simulink model "GHAME_Public"  (R2024a)
settings: Solver=ode8  StartTime=0.0  StopTime=Sim.simulation.duration  FixedStep=0.01  RelTol=1e-3
undefined symbols (not defined in the file): Data, DataPlant, IC, Sim, v0_BE_B
libraries: simulink_extras x8, simulink x1
(part 2 of 3)

== matlab function GHAME_Public/GHAME Airframe/Forces and Moments/PROPULSION/Subsystem/Updating mass and inertia ==
  data: IBBB output size=[3 3]; IBBBdot output; fmdot input; fmasse input; vmass output size=[1 1]; Sim parameter; stop_flag output
function [IBBB, IBBBdot, vmass, stop_flag] = mass(fmdot, fmasse, Sim)
% MASS  Vehicle mass and inertia as a function of expended fuel.
%
%   [IBBB, IBBBdot, vmass, stop_flag] = mass(fmdot, fmasse, Sim)
%
%   The inertia tensor is interpolated linearly between the full-tank and
%   empty-tank values according to the remaining fuel fraction.
%
%   Inputs
%     fmdot   [1x1]  Fuel mass flow (kg/s)
%     fmasse  [1x1]  Fuel mass expended since start (kg)
%     Sim     struct Vehicle mass and inertia data
%
%   Outputs
%     IBBB       [3x3]  Inertia tensor in body axes (kg m^2)
%     IBBBdot    [3x3]  Time derivative of the inertia tensor (kg m^2/s)
%     vmass      [1x1]  Current vehicle mass (kg)
%     stop_flag  [1x1]  True when the fuel is exhausted

%   Author:    Thomas Harald Müller
%   GitHub:    https://github.com/ThomasHaraldMueller
%   Copyright: (c) 2026 Thomas Harald Müller, Hamburg, Germany
%   Free to use and modify, provided this notice is kept and the author is credited.

%% Mass properties
fmass_init = Sim.vehicle.mass.fuel;          % Fuel on board at start
fmass_full = Sim.vehicle.mass.fuel_full;     % Fuel capacity
vmass_init = Sim.vehicle.mass.current;       % Total mass at start
IBBB0      = Sim.vehicle.inertia.IBBB0;      % Inertia with full tank
IBBB1      = Sim.vehicle.inertia.IBBB1;      % Inertia with empty tank

%% Mass update
% Expended fuel is limited to what was on board, so mass and inertia
% never drop below the empty-tank values
fmasse_c = min(fmasse, fmass_init);

vmass = vmass_init - fmasse_c;
fmass = fmass_init - fmasse_c;               % Remaining fuel

%% Inertia update
% Fuel fraction, 1 = full tank, 0 = empty tank
fuel_ratio = fmass / fmass_full;

dI   = IBBB0 - IBBB1;
IBBB = IBBB1 + dI * fuel_ratio;

% Chain rule, d(fuel_ratio)/dt = -fmdot/fmass_full. Zero once the tank is empty.
if fmass > 0
    IBBBdot = (-fmdot / fmass_full) * dI;
else
    IBBBdot = zeros(3);
end

%% Termination
stop_flag = (fmass <= 1e-6);

end

== matlab function GHAME_Public/GHAME Airframe/Environment/ENVIRONMENT/Wind and Turbulence/Wind Computation ==
  settings: updateMethod=CONTINUOUS
  data: Vwind input; VTAD input; VAEDS input; VAED output; Sim parameter; VAEDSD output
function [VAED, VAEDSD] = wind(Vwind, VTAD, VAEDS, Sim)
% WIND  Air velocity relative to Earth from mean wind and turbulence.
%
%   [VAED, VAEDSD] = wind(Vwind, VTAD, VAEDS, Sim)
%
%   The horizontal mean wind is smoothed by a first-order lag, so that
%   steps in the wind model do not excite the vehicle. Dryden turbulence
%   is added on top when enabled. The air-relative velocity of the vehicle
%   then follows as VBAD = VBED - VAED.
%
%   Inputs
%     Vwind   [2x1]  Mean wind [north; east] from HWM14 (m/s)
%     VTAD    [3x1]  Turbulence velocity in geodetic axes (m/s)
%     VAEDS   [3x1]  Smoothed mean wind, integrator state (m/s)
%     Sim     struct Mode switches and wind smoothing time constant
%
%   Outputs
%     VAED    [3x1]  Air velocity relative to Earth, geodetic axes (m/s)
%     VAEDSD  [3x1]  Derivative of the smoothed mean wind (m/s^2)
%
%   Initialize the VAEDS integrator with the initial wind to avoid a
%   start-up transient.

%   Author:    Thomas Harald Müller
%   GitHub:    https://github.com/ThomasHaraldMueller
%   Copyright: (c) 2026 Thomas Harald Müller, Hamburg, Germany
%   Free to use and modify, provided this notice is kept and the author is credited.

twind = Sim.wind.tau_smooth;        % Smoothing time constant (s)

VAED   = zeros(3, 1);
VAEDSD = zeros(3, 1);

% Mean wind, smoothed by a first-order lag
if Sim.mode.mwind > 0
    VAED_raw = [Vwind(1);           % North (meridional)
                Vwind(2);           % East (zonal)
                0];                 % Down, no vertical mean wind

    VAEDSD = (VAED_raw - VAEDS) / twind;
    VAED   = VAEDS;
end

% Dryden turbulence
if Sim.mode.mturb > 0
    VAED = VAED + VTAD;
end

end

== matlab function GHAME_Public/GHAME Airframe/Environment/ENVIRONMENT/Gravity Calculation ==
  data: SBII input; GRAVG output; Sim parameter
function GRAVG = cad_grav84(SBII, Sim)
% CAD_GRAV84  Gravitational acceleration with J2 in geocentric coordinates.
%
%   GRAVG = cad_grav84(SBII, Sim)
%
%   Uses the normalized second zonal harmonic C20 of the WGS84 field.
%   The geocentric frame G is north, east, down with the down axis pointing
%   to the Earth centre. The east component is zero for a zonal field.
%
%   Inputs
%     SBII    [3x1]  Position in inertial coordinates (m)
%     Sim     struct Earth constants (GM, semi-major axis, normalized C20 < 0)
%
%   Output
%     GRAVG   [3x1]  Gravitational acceleration in geocentric axes (m/s^2)

%   Author:    Thomas Harald Müller
%   GitHub:    https://github.com/ThomasHaraldMueller
%   Copyright: (c) 2026 Thomas Harald Müller, Hamburg, Germany
%   Free to use and modify, provided this notice is kept and the author is credited.

GM  = Sim.earth.GM;
a   = Sim.earth.SMAJOR_AXIS;
C20 = Sim.earth.C20;

r    = norm(SBII);
latc = asin(SBII(3) / r);           % Geocentric latitude
slat = sin(latc);
clat = cos(latc);

g0 = GM / r^2;                      % Point-mass gravity
k  = sqrt(5) * C20 * (a / r)^2;     % J2 scaling, negative for C20 < 0

% Gradient of V = GM/r * (1 + C20*(a/r)^2 * sqrt(5)/2 * (3*sin(lat)^2 - 1))
GRAVG = [ 3 * g0 * k * slat * clat;                 % North (towards equator)
          0;                                        % East
          g0 * (1 + 1.5 * k * (3 * slat^2 - 1)) ];  % Down

end

== matlab function GHAME_Public/GHAME Airframe/Forces and Moments/PROPULSION/Thrust and fuel use ==
  data: rho input; Mach input; alphax input; DVBA input; Throttle input; pdynmc input; Thrust output; fmdot output; cx_dthr output; Data parameter; Sim parameter; Throttle output; pdynmc output
function [Thrust, fmdot, cx_dthr, Throttle, pdynmc] = thrust(rho, Mach, alphax, DVBA, Throttle, pdynmc, Data, Sim)
% THRUST  Scramjet thrust, fuel mass flow and propulsive force coefficients.
%
%   [Thrust, fmdot, cx_prop, Throttle, pdynmc, cx_dthr] = thrust(rho, Mach, ...
%       alphax, DVBA, Throttle, pdynmc, Data, Sim)
%
%   The engine is modelled through the captured air mass flow. Fuel flow is
%   the stoichiometric fuel-air ratio times the equivalence ratio (Throttle)
%   times the air mass flow, and thrust follows from the specific impulse.
%
%     mdot_air  = rho * V * A_capture * acowl
%     mdot_fuel = FAR_ST * Throttle * mdot_air
%     Thrust    = Isp(Mach, Throttle) * g0 * mdot_fuel
%
%   Inputs
%     rho       [1x1]  Atmospheric density (kg/m^3)
%     Mach      [1x1]  Mach number
%     alphax    [1x1]  Angle of attack (deg)
%     DVBA      [1x1]  Airspeed (m/s)
%     Throttle  [1x1]  Commanded equivalence ratio
%     pdynmc    [1x1]  Dynamic pressure (Pa)
%     Data      struct Engine tables (Data.ThrustCoefficients)
%     Sim       struct Constants, vehicle geometry and simulation settings
%
%   Outputs
%     Thrust    [1x1]  Thrust along the body x-axis (N)
%     fmdot     [1x1]  Fuel mass flow used for the mass update (kg/s)
%     cx_prop   [1x1]  Thrust coefficient per unit throttle, T/(Throttle*q*S)
%     Throttle  [1x1]  Throttle after saturation
%     pdynmc    [1x1]  Dynamic pressure, passed through unchanged
%     cx_dthr   [1x1]  Thrust effectiveness, (dT/dThrottle)/(q*S), for the controller

%   Author:    Thomas Harald Müller
%   GitHub:    https://github.com/ThomasHaraldMueller
%   Copyright: (c) 2026 Thomas Harald Müller, Hamburg, Germany
%   Free to use and modify, provided this notice is kept and the author is credited.

%% Constants and parameters
thrtl_idle = 0.05;      % Minimum equivalence ratio
thrtl_max  = 2;         % Maximum equivalence ratio
FAR_ST     = 0.029;     % Stoichiometric fuel-air ratio (hydrogen)
dthr       = 0.05;      % Throttle step for the central difference
q_min      = 1;         % Dynamic pressure below which coefficients are set to zero (Pa)

AGRAV        = Sim.earth.AGRAV;
Sim_Extender = Sim.simulation.Sim_Extender;
acowl        = Sim.vehicle.acowl;
refa         = Sim.vehicle.geometry.refa;

%% Engine tables
Mach_vec     = Data.ThrustCoefficients.Mach_vec;
alpha_vec    = Data.ThrustCoefficients.alpha_vec;       % deg
throttle_vec = Data.ThrustCoefficients.throttle_vec;

capture_area_tab = Data.ThrustCoefficients.Capture_A;   % f(Mach, alpha)
SPI_tab          = Data.ThrustCoefficients.SPI_tab;     % f(Mach, Throttle), s

% Admissible throttle range, limited by both the engine and the table
thr_lo = max(thrtl_idle, throttle_vec(1));
thr_hi = min(thrtl_max,  throttle_vec(end));

%% Table lookups
Throttle = max(min(Throttle, thrtl_max), thrtl_idle);

% Clamp to the table range so that interp2 cannot return NaN
Mach_c  = clamp(Mach,     Mach_vec(1),  Mach_vec(end));
alpha_c = clamp(alphax,   alpha_vec(1), alpha_vec(end));
thr_c   = clamp(Throttle, thr_lo,       thr_hi);

isp = @(thr) interp2(Mach_vec, throttle_vec, SPI_tab, Mach_c, thr, 'linear');

SPI          = isp(thr_c);
capture_area = interp2(Mach_vec, alpha_vec, capture_area_tab, Mach_c, alpha_c, 'linear');

%% Thrust and fuel flow
mdot_air  = rho * DVBA * capture_area * acowl;
mdot_fuel = FAR_ST * Throttle * mdot_air;

Thrust = SPI * AGRAV * mdot_fuel;

% Testing option. Sim_Extender > 1 reduces fuel consumption to extend the
% flight time, so the mass history is only physical for Sim_Extender = 1.
fmdot = mdot_fuel / Sim_Extender;

%% Propulsive coefficients
% cx_prop is the secant T/Throttle and reproduces the thrust exactly.
% cx_dthr is the local slope dT/dThrottle, which includes the change of Isp
%
%   dT/dThrottle = g0 * FAR_ST * mdot_air * d(Isp*Throttle)/dThrottle
%
% The stencil is clamped to the table, making it one-sided at the limits.
thr_p = clamp(thr_c + dthr, thr_lo, thr_hi);
thr_m = clamp(thr_c - dthr, thr_lo, thr_hi);

dIspThr = (isp(thr_p)*thr_p - isp(thr_m)*thr_m) / (thr_p - thr_m);
dT_dthr = AGRAV * FAR_ST * mdot_air * dIspThr;

% Avoid division by zero at initialization or outside the atmosphere
qS = pdynmc * refa;
if pdynmc > q_min
    cx_prop = Thrust  / (Throttle * qS);
    cx_dthr = dT_dthr / qS;
else
    cx_prop = 0;
    cx_dthr = 0;
end

end

%% Local functions

function y = clamp(x, lo, hi)
% CLAMP  Saturate x to [lo, hi]
    y = max(min(x, hi), lo);
end

== matlab function GHAME_Public/GHAME Airframe/Environment/ENVIRONMENT/Atmosphere calculation ==
  data: rho output; press output; tempk output; vsound output; alt_km input
function [rho, press, tempk, vsound] = us76_nasa2002(alt_km)
% US76_NASA2002  1976 U.S. Standard Atmosphere from 0 to 1000 km.
%
%   [rho, press, tempk, vsound] = us76_nasa2002(alt_km)
%
%   Below 86 km the standard layers with linear temperature in geopotential
%   altitude are evaluated analytically. Above 86 km temperature follows the
%   standard piecewise model, while pressure and molecular weight are
%   interpolated quadratically (pressure in log scale) between table points.
%   Altitudes outside [0, 1000] km are clamped to the range.
%
%   Input
%     alt_km  [1x1]  Geocentric altitude (km)
%
%   Outputs
%     rho     [1x1]  Density (kg/m^3)
%     press   [1x1]  Pressure (Pa)
%     tempk   [1x1]  Temperature (K)
%     vsound  [1x1]  Speed of sound (m/s), with gamma = 1.4

%   Author:    Thomas Harald Müller
%   GitHub:    https://github.com/ThomasHaraldMueller
%   Copyright: (c) 2026 Thomas Harald Müller, Hamburg, Germany
%   Free to use and modify, provided this notice is kept and the author is credited.

%% Constants
ro  = 6356.766;     % Effective Earth radius for geopotential altitude (km)
go  = 9.80665;      % Standard gravity (m/s^2)
wmo = 28.9644;      % Sea-level molecular weight (kg/kmol)
rs  = 8314.32;      % Universal gas constant (J/(kmol K))

%% Tables
% Altitude breakpoints (km)
zs = [0, 11.019, 20.063, 32.162, 47.35, 51.413, 71.802, 86, 91, 94, ...
      97, 100, 103, 106, 108, 110, 112, 115, 120, 125, 130, 135, 140, ...
      145, 150, 155, 160, 165, 170, 180, 190, 210, 230, 265, 300, 350, ...
      400, 450, 500, 550, 600, 650, 700, 750, 800, 850, 900, 950, 1000];

% Temperature (K)
tms = [288.15, 216.65, 216.65, 228.65, 270.65, 270.65, 214.65, ...
       186.95, 186.87, 187.74, 190.40, 195.08, 202.23, 212.89, ...
       223.29, 240.00, 264.00, 300.00, 360.00, 417.23, 469.27, ...
       516.59, 559.63, 598.78, 634.39, 666.80, 696.29, 723.13, ...
       747.57, 790.07, 825.31, 878.84, 915.78, 955.20, 976.01, ...
       990.06, 995.83, 998.22, 999.24, 999.67, 999.85, 999.93, ...
       999.97, 999.99, 999.99, 1000, 1000, 1000, 1000];

% Molecular weight (kg/kmol)
wms = [28.9644, 28.9644, 28.9644, 28.9644, 28.9644, 28.9644, ...
       28.9644, 28.9522, 28.8890, 28.7830, 28.6200, 28.3950, ...
       28.1040, 27.7650, 27.5210, 27.2680, 27.0200, 26.6800, ...
       26.2050, 25.8030, 25.4360, 25.0870, 24.7490, 24.4220, ...
       24.1030, 23.7920, 23.4880, 23.1920, 22.9020, 22.3420, ...
       21.8090, 20.8250, 19.9520, 18.6880, 17.7260, 16.7350, ...
       15.9840, 15.2470, 14.3300, 13.0920, 11.5050, 9.7180, ...
       7.9980, 6.5790, 5.5430, 4.8490, 4.4040, 4.1220, 3.9400];

% Pressure (tabulated in hPa, converted to Pa)
ps = [1013.25, 226.32, 54.7487, 8.68014, 1.10905, 0.66938, ...
      0.039564, 3.7338e-03, 1.5381e-03, 9.0560e-04, 5.3571e-04, ...
      3.2011e-04, 1.9742e-04, 1.2454e-04, 9.3188e-05, 7.1042e-05, ...
      5.5547e-05, 4.0096e-05, 2.5382e-05, 1.7354e-05, 1.2505e-05, ...
      9.3568e-06, 7.2028e-06, 5.6691e-06, 4.5422e-06, 3.6930e-06, ...
      3.0395e-06, 2.5278e-06, 2.1210e-06, 1.5271e-06, 1.1266e-06, ...
      6.4756e-07, 3.9276e-07, 1.7874e-07, 8.7704e-08, 3.4498e-08, ...
      1.4518e-08, 6.4468e-09, 3.0236e-09, 1.5137e-09, 8.2130e-10, ...
      4.8865e-10, 3.1908e-10, 2.2599e-10, 1.7036e-10, 1.3415e-10, ...
      1.0873e-10, 8.9816e-11, 7.5138e-11] * 100;

%% Layer index
alt_km = min(max(alt_km, 0), 1000);
n = numel(zs);

% Interval i with zs(i) <= alt_km < zs(i+1), limited to the last interval.
% A plain loop keeps i a fixed-size scalar for code generation.
i = 1;
while i < n - 1 && zs(i+1) <= alt_km
    i = i + 1;
end

%% Layers 1 to 7 (0 to 86 km), analytic in geopotential altitude
if i <= 7
    zl = ro * zs(i)   / (ro + zs(i));       % Geopotential altitudes (km)
    zu = ro * zs(i+1) / (ro + zs(i+1));
    ht = ro * alt_km  / (ro + alt_km);

    lapse = (tms(i+1) - tms(i)) / (zu - zl);   % Temperature gradient (K/km)
    tempk = tms(i) + lapse * (ht - zl);
    wm    = wmo;

    if abs(lapse) > 1e-12
        press = ps(i) * (tms(i) / tempk)^(go * wmo / (rs * lapse * 1e-3));
    else
        press = ps(i) * exp(-go * wmo * (ht - zl) * 1e3 / (rs * tms(i)));
    end

%% Layers above 86 km, standard temperature model and table interpolation
else
    if i == 8                       % 86 to 91 km, isothermal at 186.87 K
        tempk = tms(9);
    elseif i <= 15                  % 91 to 110 km, elliptical
        tempk = 263.1905 - 76.3232 * sqrt(1 - ((alt_km - 91) / 19.9429)^2);
    elseif i <= 18                  % 110 to 120 km, linear
        tempk = 240 + 12 * (alt_km - 110);
    else                            % Above 120 km, exponential
        xi    = (alt_km - 120) * (ro + 120) / (ro + alt_km);
        tempk = 1000 - 640 * exp(-0.01875 * xi);
    end

    % Quadratic interpolation over the interval and its upper neighbour
    j = i;
    if i == n - 1
        j = i - 1;                  % Keep the stencil inside the table
    end
    [wma, lpa] = lagrange3(zs, wms, log(ps), j, alt_km);
    wmb = wma;
    lpb = lpa;

    % Average with the stencil shifted one point down, except at the ends
    if i ~= 8 && i ~= n - 1
        [wmb, lpb] = lagrange3(zs, wms, log(ps), j - 1, alt_km);
    end

    press = exp((lpa + lpb) / 2);
    wm    = (wma + wmb) / 2;
end

%% Density and speed of sound
rho    = wm * press / (rs * tempk);
vsound = sqrt(1.4 * press / rho);

end

%% Local functions

function [y1, y2] = lagrange3(z, f1, f2, j, x)
% LAGRANGE3  Quadratic Lagrange interpolation of two tables through the
%   points j, j+1 and j+2.
    z0 = z(j);  z1 = z(j+1);  z2 = z(j+2);
    L0 = (x - z1) * (x - z2) / ((z0 - z1) * (z0 - z2));
    L1 = (x - z0) * (x - z2) / ((z1 - z0) * (z1 - z2));
    L2 = (x - z0) * (x - z1) / ((z2 - z0) * (z2 - z1));
    y1 = f1(j) * L0 + f1(j+1) * L1 + f1(j+2) * L2;
    y2 = f2(j) * L0 + f2(j+1) * L1 + f2(j+2) * L2;
end
